simulink model "snap_sys_clk_feng"  (R2019a)
settings: Solver=VariableStepDiscrete  StartTime=0.0  StopTime=10.0  RelTol=1e-3
undefined symbols (not defined in the file): datetime, posixtime
libraries: xbsIndex_r4 x5252, casper_library_misc x69, xps_library x6, casper_library_delays x3
(part 1 of 45)
settings Model: Creator=jackh  LastModifiedBy=jackh
settings DataIOCC: ReturnWorkspaceOutputs=off
settings OptimizationCC: DefaultParameterBehavior=Inlined
settings DebuggingCC: ArithmeticOperatorsInVariantConditions=warning
settings SFSimCC: SimUseLocalCustomCode=off
settings RTWCC: RTWUseLocalCustomCode=off
settings CodeAppCC: StateflowObjectComments=on

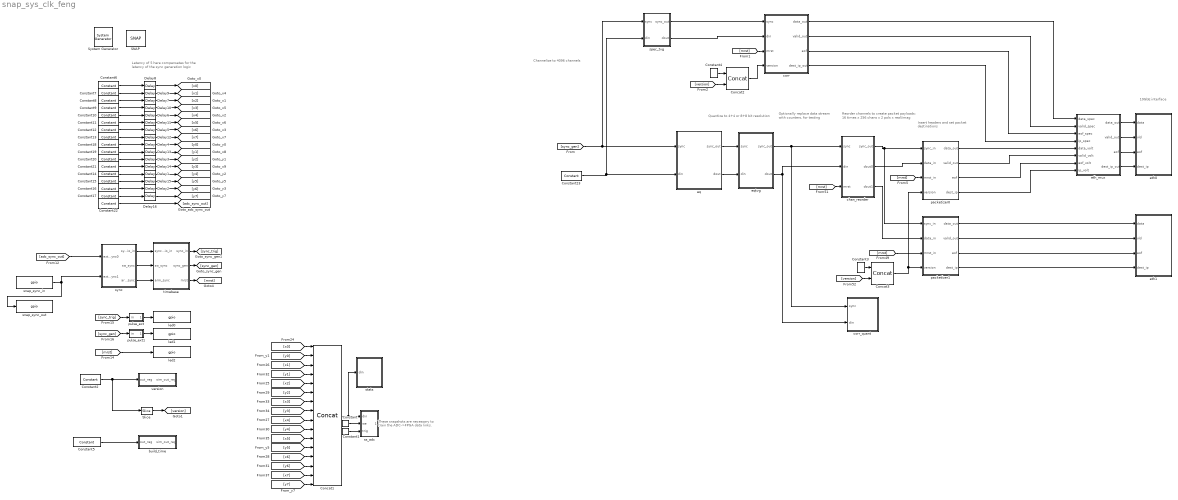
== system snap_sys_clk_feng ==
  note: 10GbE interface
  note: Insert headers and
      | set packet destinations
  note: Reorder channels to
      | create packet payloads:
      | 16 times x 256 chans x 2 pols x real/imag
  note: Optionally replace data
      | stream with counters, for testing
  note: Quantize to 4+4 or 8+8 bit resolution
  note: Channelize to 4096 channels
  note: These snapshots are necessary
      | to train the ADC->FPGA data links.
  note: Latency of 5 here compensates
      | for the latency of the sync generation logic
  " System Generator" : xbsIndex_r4/ System Generator  Tag=genX  xilinxfamily=kintex7  part=xc7k160t  speed=-2  package=ffg676  synthesis_tool=XST  clock_wrapper=Clock Enables  directory=/home/jackh/src/ata_snap/snap_sys_clk_feng/sysgen  proj_type=Vivado  Synth_file=Vivado Synthesis Defaults  Impl_file=Vivado Implementation Defaults  testbench=off  simulink_period=1  sysclk_period=10  dcm_input_clock_period=10  incr_netlist=off  trim_vbits=Everywhere in SubSystem  dbl_ovrd=According to Block Masks  core_generation=According to Block Masks  run_coregen=off  deprecated_control=off  eval_field=0  block_type=sysgen
  Concat1 : xbsIndex_r4/Concat  num_inputs=16  dbl_ovrd=off  block_type=concat
  Concat2 : xbsIndex_r4/Concat  num_inputs=2  dbl_ovrd=off  block_type=concat
  Concat3 : xbsIndex_r4/Concat  num_inputs=2  dbl_ovrd=off  block_type=concat
  Constant : xbsIndex_r4/Constant  const=0  gui_display_data_type=Boolean  arith_type=Boolean  n_bits=16  bin_pt=14  preci_type=Single  exp_width=8  frac_width=24  explicit_period=on  period=1  equ=P=C  opselect=C  inp2=PCIN>>17  opr=+  inp1=P  carry=CIN  dbl_ovrd=off  block_type=constant
  Constant1 : xbsIndex_r4/Constant  const=0  gui_display_data_type=Boolean  arith_type=Boolean  n_bits=16  bin_pt=14  preci_type=Single  exp_width=8  frac_width=24  explicit_period=on  period=1  equ=P=C  opselect=C  inp2=PCIN>>17  opr=+  inp1=P  carry=CIN  dbl_ovrd=off  block_type=constant
  Constant{6..21} (16 alike) : xbsIndex_r4/Constant  const=0  gui_display_data_type=Fixed-point  arith_type=Unsigned  n_bits=8  bin_pt=0  preci_type=Single  exp_width=8  frac_width=24  explicit_period=on  period=1  equ=P=C  opselect=C  inp2=PCIN>>17  opr=+  inp1=P  carry=CIN  dbl_ovrd=off  block_type=constant
  Constant2 : xbsIndex_r4/Constant  const=((2^6 + 2^5 + 0)*2^8) + 0  gui_display_data_type=Fixed-point  arith_type=Unsigned  n_bits=7+8  bin_pt=0  preci_type=Single  exp_width=8  frac_width=24  explicit_period=on  period=1  equ=P=C  opselect=C  inp2=PCIN>>17  opr=+  inp1=P  carry=CIN  dbl_ovrd=off  block_type=constant
  Constant22 : xbsIndex_r4/Constant  const=0  gui_display_data_type=Boolean  arith_type=Boolean  n_bits=8  bin_pt=7  preci_type=Single  exp_width=8  frac_width=24  explicit_period=on  period=1  equ=P=C  opselect=C  inp2=PCIN>>17  opr=+  inp1=P  carry=CIN  dbl_ovrd=off  block_type=constant
  Constant23 : xbsIndex_r4/Constant  const=0  gui_display_data_type=Fixed-point  arith_type=Unsigned  n_bits=400  bin_pt=0  preci_type=Single  exp_width=8  frac_width=24  explicit_period=on  period=1  equ=P=C  opselect=C  inp2=PCIN>>17  opr=+  inp1=P  carry=CIN  dbl_ovrd=off  block_type=constant
  Constant3 : xbsIndex_r4/Constant  const=1  gui_display_data_type=Fixed-point  arith_type=Unsigned  n_bits=1  bin_pt=0  preci_type=Single  exp_width=8  frac_width=24  explicit_period=on  period=1  equ=P=C  opselect=C  inp2=PCIN>>17  opr=+  inp1=P  carry=CIN  dbl_ovrd=off  block_type=constant
  Constant4 : xbsIndex_r4/Constant  const=0  gui_display_data_type=Fixed-point  arith_type=Unsigned  n_bits=1  bin_pt=0  preci_type=Single  exp_width=8  frac_width=24  explicit_period=on  period=1  equ=P=C  opselect=C  inp2=PCIN>>17  opr=+  inp1=P  carry=CIN  dbl_ovrd=off  block_type=constant
  Constant5 : xbsIndex_r4/Constant  const=int32(posixtime(datetime('now')))  gui_display_data_type=Fixed-point  arith_type=Unsigned  n_bits=32  bin_pt=0  preci_type=Single  exp_width=8  frac_width=24  explicit_period=on  period=1  equ=P=C  opselect=C  inp2=PCIN>>17  opr=+  inp1=P  carry=CIN  dbl_ovrd=off  block_type=constant
  Delay{1..16} (16 alike) : xbsIndex_r4/Delay  rst=off  infoeditControl=Selection of Reset will increase slice count due to use of real FFs and instead of SRLs  en=off  latency=5  reg_retiming=off  dbl_ovrd=off  block_type=delay
      settings: block_version=11.4
  SNAP : xps_library/Platforms/SNAP  Tag=xps:xsg  hw_sys=SNAP:xc7k160t  clk_src=sys_clk  clk_rate=100  use_microblaze=on  sample_period=1  synthesis_tool=XST
      settings: SourceProductName=CASPER XPS Blockset
  Slice : xbsIndex_r4/Slice  nbits=7  boolean_output=off  mode=Lower Bit Location + Width  bit1=0  base1=MSB of Input  bit0=8  base0=LSB of Input  dbl_ovrd=off  block_type=slice
  build_time : Subsystem  Tag=xps:sw_reg  AncestorBlock=xps_library/Memory/software_register  mask(swreg){io_dir=To Processor, io_delay=0, init_val=0, sample_period=1, names=reg, bitwidths=32, bin_pts=0, arith_types=0, sim_port=on, show_format=on}
      mask prompts: io_dir "I/O direction"; io_delay "I/O delay"; init_val "Initial Value"; sample_period "Sample period"; names "Bitfield names [msb...lsb]"; bitwidths "Bitfield widths"; bin_pts "Bitfield binary pts"; arith_types "Bitfield types, ufix=0, fix=1, bool=2"; sim_port "Provide sim input/output?"; show_format "Print format string?"
      mask help: A 32-bit software-accessible register. Can be divided into bitfields of varying widths and types using the fields in the block mask.
      mask init:
      | swreg_init(gcb)
      settings: AttributesFormatString=1output:uf32.0 = 32 bits
      mask TypeOptions io_dir: To Processor | From Processor
      mask Callback io_dir:
      | mask_enables = get_param(gcb, 'MaskEnables');
      | mask_names = get_param(gcb, 'MaskNames');
      | if strcmp(get_param(gcb, 'io_dir'), 'To Processor'),
      |     mask_enables{ismember(mask_names, 'sample_period')} = 'off';
      | else
      |     mask_enables{ismember(mask_names, 'sample_period')} = 'on';
      | end
      | set_param(gcb, 'MaskEnables', mask_enables);
      mask DialogControl ParameterTabVar0 Prompt: Setup
  chan_reorder : Subsystem
  corr : Subsystem  mask{n_chan_bits=12}
      mask prompts: n_chan_bits "Number of channels? (2^?)"
  corr_quant : Subsystem  mask{n_chan_bits=12}
      mask prompts: n_chan_bits "Number of channels? (2^?)"
  eq : Subsystem
  eqtvg : Subsystem
  eth0 : Subsystem
  eth1 : Subsystem
  eth_mux : Subsystem
  led0 : xps_library/IO/gpio  Tag=xps:gpio  io_group_params_forwarded=on  io_group=ROACH:led  io_group_real=led  io_group_custom=0  io_dir=out  arith_type=Boolean  bitwidth=1  bin_pt=0  bit_index=0  sample_period=1  use_single_ended=off  use_ddr=off  reg_iob=on  reg_clk_phase=0  termination=None
      settings: SourceProductName=CASPER XPS Blockset
  led1 : xps_library/IO/gpio  Tag=xps:gpio  io_group_params_forwarded=on  io_group=ROACH:led  io_group_real=led  io_group_custom=0  io_dir=out  arith_type=Boolean  bitwidth=1  bin_pt=0  bit_index=1  sample_period=1  use_single_ended=off  use_ddr=off  reg_iob=on  reg_clk_phase=0  termination=None
      settings: SourceProductName=CASPER XPS Blockset
  led2 : xps_library/IO/gpio  Tag=xps:gpio  io_group_params_forwarded=on  io_group=ROACH:led  io_group_real=led  io_group_custom=0  io_dir=out  arith_type=Boolean  bitwidth=1  bin_pt=0  bit_index=2  sample_period=1  use_single_ended=off  use_ddr=off  reg_iob=on  reg_clk_phase=0  termination=None
      settings: SourceProductName=CASPER XPS Blockset
  packetizer0 : Subsystem  mask{nchan_bits=12, npol_bits=4+1, nparallel_bits=3, step_bits=5, time_step_bits=4}
      mask prompts: nchan_bits "Number of channels (including unsent) (2^?)"; npol_bits "Number of pols (2^?)"; nparallel_bits "Parallel samples (2^?)"; step_bits "Step granularity (2^?)"; time_step_bits "Time Steps per cycle (2^?)"
  packetizer1 : Subsystem  mask{nchan_bits=12, npol_bits=4+1, nparallel_bits=3, step_bits=5, time_step_bits=4}
      mask prompts: nchan_bits "Number of channels (including unsent) (2^?)"; npol_bits "Number of pols (2^?)"; nparallel_bits "Parallel samples (2^?)"; step_bits "Step granularity (2^?)"; time_step_bits "Time Steps per cycle (2^?)"
  pulse_ext : Subsystem  AncestorBlock=casper_library_misc/pulse_ext  mask(pulse_ext){pulse_len=2^25}
      mask prompts: pulse_len "Length of Pulse"
      mask help:
      | Extends a boolean signal to be high for the specified number of clocks after
      | the last high input.
      mask init:
      | bits = ceil(log2(pulse_len+1));
      mask Help: eval('xlWeb(''http://casper.berkeley.edu/wiki/Pulse_ext'')')
  pulse_ext1 : Subsystem  AncestorBlock=casper_library_misc/pulse_ext  mask(pulse_ext){pulse_len=2^25}
      mask prompts: pulse_len "Length of Pulse"
      mask help:
      | Extends a boolean signal to be high for the specified number of clocks after
      | the last high input.
      mask init:
      | bits = ceil(log2(pulse_len+1));
      mask Help: eval('xlWeb(''http://casper.berkeley.edu/wiki/Pulse_ext'')')
  snap_sync_in : xps_library/IO/gpio  Tag=xps:gpio  io_group_params_forwarded=on  io_group=ROACH:led  io_group_real=sync_in  io_group_custom=0  io_dir=in  arith_type=Boolean  bitwidth=1  bin_pt=0  bit_index=0  sample_period=1  use_single_ended=off  use_ddr=off  reg_iob=on  reg_clk_phase=0  termination=None
      settings: SourceProductName=CASPER XPS Blockset
  snap_sync_out : xps_library/IO/gpio  Tag=xps:gpio  io_group_params_forwarded=on  io_group=ROACH:led  io_group_real=sync_out  io_group_custom=0  io_dir=out  arith_type=Boolean  bitwidth=1  bin_pt=0  bit_index=0  sample_period=1  use_single_ended=on  use_ddr=off  reg_iob=on  reg_clk_phase=0  termination=None
      settings: SourceProductName=CASPER XPS Blockset
  spec_tvg : Subsystem
  ss_adc : Subsystem  Tag=casper:snapshot  AncestorBlock=casper_library_scopes/snapshot  mask(snapshot){storage=bram, dram_dimm=1, dram_clock=200, nsamples=9, data_width=128, offset=off, circap=off, value=off, ext_arm=off, ext_circ=off, provide_outputs=on, use_dsp48=off}
      mask prompts: storage "Storage medium"; dram_dimm "DRAM dimm"; dram_clock "DRAM clock rate"; nsamples "Number of Samples (2^?)"; data_width "Data width"; offset "Start delay support"; circap "Circular capture support"; value "Extra value capture support"; ext_arm "External arm support"; ext_circ "External circular capture support"; provide_outputs "Provide outputs"; use_dsp48 "Use DSP48s to implement counters"
      mask help:
      | Standard snap block, but with the following optional extras;
      |  1) Optionally delay the fabric trigger by a user-specified number of valids.
      |  2) Capture continuously after a trigger until a stop pulse is received. Data is captured into BRAM continuously, with old data being overwritten until a stop command is received. Then stop capturing when memory is filled. This enables you to get some data before and some data after the stop pulse. Use the 'tr_en_cnt' register to determine where you are in your vector. 'Addr' register's MSb now indicates 'busy capturing'.
      |  3) Optionally capture a value on an input port to a register at the same time as the first data sample.
      |  4) Implement counters using DSP48Es to save resources.
      mask init:
      | snapshot_init(gcb, ...
      |     'storage', storage, ...
      |     'dram_dimm', dram_dimm, ...
      |     'dram_clock', dram_clock, ...
      |     'nsamples', nsamples, ...
      |     'data_width', data_width, ...
      |     'offset', offset, ...
      |     'circap', circap, ...
      |     'value', value, ...
      |     'ext_arm', ext_arm, ...
      |     'ext_circ', ext_circ, ...
      |     'provide_outputs', 'off', ...
      |     'use_dsp48', use_dsp48);
      settings: AttributesFormatString=|
      | 128 wide, 512 deep
      | debugID: 6419356
      mask TypeOptions storage: bram | dram
      mask Callback storage: snapshot_callback();
      mask TypeOptions dram_dimm: 1 | 2 | 3 | 4
      mask TypeOptions dram_clock: 200 | 250 | 266 | 300 | 333
      mask TypeOptions data_width: 8 | 16 | 32 | 64 | 128
  stats : Subsystem
  sync : Subsystem
  timebase : Subsystem
  version : Subsystem  Tag=xps:sw_reg  AncestorBlock=xps_library/Memory/software_register  mask(swreg){io_dir=To Processor, io_delay=0, init_val=0, sample_period=1, names=reg, bitwidths=7+8, bin_pts=0, arith_types=0, sim_port=on, show_format=on}
      mask prompts: io_dir "I/O direction"; io_delay "I/O delay"; init_val "Initial Value"; sample_period "Sample period"; names "Bitfield names [msb...lsb]"; bitwidths "Bitfield widths"; bin_pts "Bitfield binary pts"; arith_types "Bitfield types, ufix=0, fix=1, bool=2"; sim_port "Provide sim input/output?"; show_format "Print format string?"
      mask help: A 32-bit software-accessible register. Can be divided into bitfields of varying widths and types using the fields in the block mask.
      mask init:
      | swreg_init(gcb)
      settings: AttributesFormatString=1output:uf15.0 = 15 bits
      mask TypeOptions io_dir: To Processor | From Processor
      mask Callback io_dir:
      | mask_enables = get_param(gcb, 'MaskEnables');
      | mask_names = get_param(gcb, 'MaskNames');
      | if strcmp(get_param(gcb, 'io_dir'), 'To Processor'),
      |     mask_enables{ismember(mask_names, 'sample_period')} = 'off';
      | else
      |     mask_enables{ismember(mask_names, 'sample_period')} = 'on';
      | end
      | set_param(gcb, 'MaskEnables', mask_enables);
      mask DialogControl ParameterTabVar0 Prompt: Setup
  wires:
  sync/1(sync_gpio_in) -> timebase/1(sync_gpio_in)
  sync/2(sw_sync) -> timebase/2(sw_sync)
  sync/3(arm_sync) -> timebase/3(arm_sync)
  timebase/2(sync_gen) -> [sync_gen]
  timebase/1(sync_in) -> [sync_trig]
  timebase/3(mrst) -> [mrst]
  [adc_sync_out] -> sync/1(ext_sync0)
  [mrst] -> led2/1
  pulse_ext/1(out) -> led0/1
  pulse_ext1/1(out) -> led1/1
  [sync_trig] -> pulse_ext/1(in)
  [sync_gen] -> pulse_ext1/1(in)
  Delay2/1 -> [y6]
  Delay1/1 -> [y4]
  Delay3/1 -> [y2]
  Delay4/1 -> [y0]
  Delay5/1 -> [x6]
  Delay6/1 -> [x4]
  Delay7/1 -> [x2]
  Delay8/1 -> [x0]
  Concat1/1 -> stats/1(din), ss_adc/1(din)
  Constant/1 -> ss_adc/2(we)
  Constant1/1 -> ss_adc/3(trig)
  Delay9/1 -> [x1]
  Delay10/1 -> [x3]
  Delay11/1 -> [x5]
  Delay12/1 -> [x7]
  Delay13/1 -> [y1]
  Delay14/1 -> [y3]
  Delay15/1 -> [y5]
  Delay16/1 -> [y7]
  [x0] -> Concat1/1
  [y0] -> Concat1/2
  [x2] -> Concat1/5
  [y2] -> Concat1/6
  [x4] -> Concat1/9
  [y4] -> Concat1/10
  [x6] -> Concat1/13
  [x1] -> Concat1/3
  [y1] -> Concat1/4
  [x3] -> Concat1/7
  [y3] -> Concat1/8
  [x5] -> Concat1/11
  [y5] -> Concat1/12
  [y6] -> Concat1/14
  [x7] -> Concat1/15
  [y7] -> Concat1/16
  Constant23/1 -> spec_tvg/2(din), eq/2(din)
  [sync_gen] -> spec_tvg/1(sync), eq/1(sync)
  eq/1(sync_out) -> eqtvg/1(sync)
  eq/2(dout) -> eqtvg/2(din)
  eqtvg/1(sync_out) -> chan_reorder/1(sync), corr_quant/1(sync)
  eqtvg/2(dout) -> chan_reorder/2(din), corr_quant/2(din)
  chan_reorder/1(sync_out) -> packetizer1/1(sync_in), packetizer0/1(sync_in)
  chan_reorder/2(dout0) -> packetizer0/2(data_in)
  [mrst] -> corr/3(mrst)
  corr/1(data_out) -> eth_mux/1(data_spec)
  corr/2(valid_out) -> eth_mux/2(valid_spec)
  corr/3(eof) -> eth_mux/3(eof_spec)
  corr/4(dest_ip_out) -> eth_mux/4(ip_spec)
  eth_mux/1(data_out) -> eth0/1(data)
  eth_mux/2(valid_out) -> eth0/2(vld)
  eth_mux/3(eof) -> eth0/3(eof)
  eth_mux/4(dest_ip_out) -> eth0/4(dest_ip)
  Constant2/1 -> version/1(out_reg), Slice/1
  Slice/1 -> [version]
  Constant4/1 -> Concat2/1
  [version] -> Concat2/2
  Concat2/1 -> corr/4(version)
  spec_tvg/1(sync_out) -> corr/1(sync)
  spec_tvg/2(dout) -> corr/2(din)
  Constant6/1 -> Delay8/1
  Constant7/1 -> Delay9/1
  Constant8/1 -> Delay7/1
  Constant9/1 -> Delay10/1
  Constant10/1 -> Delay6/1
  Constant11/1 -> Delay11/1
  Constant12/1 -> Delay5/1
  Constant13/1 -> Delay12/1
  Constant18/1 -> Delay4/1
  Constant19/1 -> Delay13/1
  Constant20/1 -> Delay3/1
  Constant21/1 -> Delay14/1
  Constant14/1 -> Delay1/1
  Constant15/1 -> Delay15/1
  Constant16/1 -> Delay2/1
  Constant17/1 -> Delay16/1
  Constant22/1 -> [adc_sync_out]
  snap_sync_in/1 -> snap_sync_out/1, sync/2(ext_sync1)
  Constant5/1 -> build_time/1(out_reg)
  [mrst] -> chan_reorder/3(mrst)
  packetizer0/1(data_out) -> eth_mux/5(data_volt)
  packetizer0/2(valid_out) -> eth_mux/6(valid_volt)
  packetizer0/3(eof) -> eth_mux/7(eof_volt)
  packetizer0/4(dest_ip) -> eth_mux/8(ip_volt)
  [mrst] -> packetizer0/3(mrst_in)
  Concat3/1 -> packetizer1/4(version), packetizer0/4(version)
  packetizer1/1(data_out) -> eth1/1(data)
  packetizer1/2(valid_out) -> eth1/2(vld)
  packetizer1/3(eof) -> eth1/3(eof)
  packetizer1/4(dest_ip) -> eth1/4(dest_ip)
  [mrst] -> packetizer1/3(mrst_in)
  chan_reorder/3(dout1) -> packetizer1/2(data_in)
  Constant3/1 -> Concat3/1
  [version] -> Concat3/2

== system snap_sys_clk_feng/build_time ==
  out_reg : Inport
  assert_reg : xbsIndex_r4/Assert  assert_type=on  type_source=Explicitly  gui_display_data_type=Fixed-point  arith_type=Unsigned  n_bits=32  bin_pt=0  preci_type=Single  exp_width=8  frac_width=24  assert_rate=off  rate_source=Explicitly  period=1  output_port=on  block_type=assert
  cast_gw : xbsIndex_r4/Convert  gui_display_data_type=Fixed-point  arith_type=Unsigned  n_bits=32  bin_pt=0  float_type=Single  exp_bits=8  fraction_bits=24  quantization=Truncate  overflow=Wrap  en=off  latency=1  pipeline=off  dbl_ovrd=off  block_type=convert
  io_delay : xbsIndex_r4/Delay  rst=off  infoeditControl=Selection of Reset will increase slice count due to use of real FFs and instead of SRLs  en=off  latency=0  reg_retiming=on  dbl_ovrd=off  block_type=delay
  reint1 : xbsIndex_r4/Reinterpret  force_arith_type=on  arith_type=Unsigned  force_bin_pt=on  bin_pt=0  block_type=reinterpret
  sim_out : Terminator
  sim_out_reg_gw : xbsIndex_r4/Gateway Out  inherit_from_input=off  hdl_port=off  rows=1  columns=1  UseAsDAC=off  DACChannel='1'  interface=None  automatic_assignment=on  address_offset=hex2dec('00')  intf_name=''  intf_description=''  timing_constraint=None  locs_specified=off  LOCs={}  io_standard={}  block_type=gatewayout
  sim_out_reg_sim_delay : xbsIndex_r4/Delay  rst=off  infoeditControl=Selection of Reset will increase slice count due to use of real FFs and instead of SRLs  en=off  latency=1  reg_retiming=on  dbl_ovrd=off  block_type=delay
  snap_sys_clk_feng_build_time_user_data_in : xbsIndex_r4/Gateway Out  inherit_from_input=off  hdl_port=on  rows=1  columns=1  UseAsDAC=off  DACChannel='1'  interface=None  automatic_assignment=on  address_offset=hex2dec('00')  intf_name=''  intf_description=''  timing_constraint=None  locs_specified=off  LOCs={}  io_standard={}  block_type=gatewayout
  sim_out_reg : Outport
  wires:
  sim_out_reg_sim_delay/1 -> sim_out_reg_gw/1
  sim_out_reg_gw/1 -> sim_out_reg/1
  io_delay/1 -> cast_gw/1
  cast_gw/1 -> snap_sys_clk_feng_build_time_user_data_in/1
  snap_sys_clk_feng_build_time_user_data_in/1 -> sim_out/1
  out_reg/1 -> sim_out_reg_sim_delay/1, assert_reg/1
  assert_reg/1 -> reint1/1
  reint1/1 -> io_delay/1

== system snap_sys_clk_feng/chan_reorder ==
  note: in 4-bit mode -- slice the bits we care about
      | and send them to both packetizers.
      |
      | in 8 bit mode, split frequencies
  note: Only allow one sync after MRST.
      | This is because we don't know the appropriate
      | reorder orders for non-double-buffered runtime-configuratble
      | reorders
  note: input: 16 times x 1024 chans x 4 chans(parallel) x 2 pols
      |
      | output:
      | 1024 chans x 16 times x 4 chans (parallel) x 2 pols
      |
      | OR
      |
      | Nc x 16 times x 1024/Nc chans x 4 chans (parallel) x 2 pols
  note: reorder serial channels
      | so channels which we don't care about
      | can be placed in convenient
      | place to facilitate inter-packet gaps
  note: Reorder each parallel 64 bits to combine polarizations:
      |
      | order is now:
      |
      | serial_chans (1024) x parallel_chans (4) x pols (2)
  note: Use this programmable
      | map to mess with the channel
      | ordering.
      |
      | This lets us interleave channels we want to send, with channels
      | we don't care about, allowing the data rate to be kept below 10Gb/s
      |
      | Input is 4 channels x 2 pols in parallel.
      | Over 1024 clocks we get a full spectrum for these inputs.
  note: output:
      | 4096 chans x 4 times x 4 time (parallel) x 2 pols
  sync : Inport
  din : Inport  Port=2
  mrst : Inport  Port=3
  Constant4 : xbsIndex_r4/Constant  const=1.0  gui_display_data_type=Boolean  arith_type=Boolean  n_bits=16  bin_pt=14  preci_type=Single  exp_width=8  frac_width=24  explicit_period=on  period=1  equ=P=C  opselect=C  inp2=PCIN>>17  opr=+  inp1=P  carry=CIN  dbl_ovrd=off  block_type=constant
  Delay : xbsIndex_r4/Delay  rst=off  infoeditControl=Selection of Reset will increase slice count due to use of real FFs and instead of SRLs  en=off  latency=1  reg_retiming=off  dbl_ovrd=off  block_type=delay
  Delay1 : xbsIndex_r4/Delay  rst=off  infoeditControl=Selection of Reset will increase slice count due to use of real FFs and instead of SRLs  en=off  latency=1  reg_retiming=off  dbl_ovrd=off  block_type=delay
  Delay2 : xbsIndex_r4/Delay  rst=off  infoeditControl=Selection of Reset will increase slice count due to use of real FFs and instead of SRLs  en=off  latency=1  reg_retiming=off  dbl_ovrd=off  block_type=delay
  Inverter : xbsIndex_r4/Inverter  en=off  latency=0  dbl_ovrd=off  block_type=inv
  Logical : xbsIndex_r4/Logical  logical_function=AND  inputs=2  en=off  latency=0  precision=Full  arith_type=Unsigned  n_bits=16  bin_pt=0  align_bp=on  dbl_ovrd=off  block_type=logical
  Mux2 : xbsIndex_r4/Mux  inputs=2  en=off  latency=1  precision=Full  arith_type=Unsigned  n_bits=16  bin_pt=14  quantization=Truncate  overflow=Wrap  dbl_ovrd=off  block_type=mux
  Mux3 : xbsIndex_r4/Mux  inputs=2  en=off  latency=1  precision=Full  arith_type=Unsigned  n_bits=16  bin_pt=14  quantization=Truncate  overflow=Wrap  dbl_ovrd=off  block_type=mux
  Mux5 : xbsIndex_r4/Mux  inputs=2  en=off  latency=1  precision=Full  arith_type=Unsigned  n_bits=16  bin_pt=14  quantization=Truncate  overflow=Wrap  dbl_ovrd=off  block_type=mux
  Register : xbsIndex_r4/Register  init=0  rst=on  en=on  dbl_ovrd=off  block_type=register
  demux : Subsystem
  gpu_weird_order : Subsystem  Tag=xps:sw_reg  AncestorBlock=xps_library/Memory/software_register  mask(swreg){io_dir=From Processor, io_delay=0, init_val=0, sample_period=1, names=reg, bitwidths=1, bin_pts=0, arith_types=0, sim_port=on, show_format=on}
      mask prompts: io_dir "I/O direction"; io_delay "I/O delay"; init_val "Initial Value"; sample_period "Sample period"; names "Bitfield names [msb...lsb]"; bitwidths "Bitfield widths"; bin_pts "Bitfield binary pts"; arith_types "Bitfield types, ufix=0, fix=1, bool=2"; sim_port "Provide sim input/output?"; show_format "Print format string?"
      mask help: A 32-bit software-accessible register. Can be divided into bitfields of varying widths and types using the fields in the block mask.
      mask init:
      | swreg_init(gcb)
      settings: AttributesFormatString=1input:uf1.0 = 1 bits
      mask TypeOptions io_dir: To Processor | From Processor
      mask Callback io_dir:
      | mask_enables = get_param(gcb, 'MaskEnables');
      | mask_names = get_param(gcb, 'MaskNames');
      | if strcmp(get_param(gcb, 'io_dir'), 'To Processor'),
      |     mask_enables{ismember(mask_names, 'sample_period')} = 'off';
      | else
      |     mask_enables{ismember(mask_names, 'sample_period')} = 'on';
      | end
      | set_param(gcb, 'MaskEnables', mask_enables);
      mask DialogControl ParameterTabVar0 Prompt: Setup
  parallel_reorder1 : Subsystem
  reorder3 : Subsystem  AncestorBlock=casper_library_reorder/reorder  mask(reorder){map=reshape(permute(reshape([0:1024*16 - 1], 1024, 16), [2,1]), 1024*16, 1), n_bits=2*4*16, n_inputs=1, bram_latency=2, map_latency=2, fanout_latency=2, double_buffer=0, bram_map=on, software_controlled=off}
      mask prompts: map "Output Order:"; n_bits "Data width in"; n_inputs "Number of inputs"; bram_latency "BRAM Latency"; map_latency "Map Latency"; fanout_latency "Fanout latency"; double_buffer "Double Buffer"; bram_map "Use BlockRAM for Map"; software_controlled "Use runtime software control"
      mask init:
      | reorder_init(gcb, ...
      |     'map', map, ...
      |     'n_bits', n_bits, ...
      |     'n_inputs', n_inputs, ...
      |     'bram_latency', bram_latency, ...
      |     'map_latency', map_latency, ...
      |     'fanout_latency', fanout_latency, ...
      |     'double_buffer', double_buffer, ...
      |     'bram_map', bram_map, ...
      |     'software_controlled', software_controlled);
      settings: AttributesFormatString=order=7
      mask Help: eval('xlWeb(''http://casper.berkeley.edu/wiki/Reorder'')')
  skip_c_t_transpose : Subsystem  Tag=xps:sw_reg  AncestorBlock=xps_library/Memory/software_register  mask(swreg){io_dir=From Processor, io_delay=0, init_val=0, sample_period=1, names=reg, bitwidths=1, bin_pts=0, arith_types=0, sim_port=on, show_format=on}
      mask prompts: io_dir "I/O direction"; io_delay "I/O delay"; init_val "Initial Value"; sample_period "Sample period"; names "Bitfield names [msb...lsb]"; bitwidths "Bitfield widths"; bin_pts "Bitfield binary pts"; arith_types "Bitfield types, ufix=0, fix=1, bool=2"; sim_port "Provide sim input/output?"; show_format "Print format string?"
      mask help: A 32-bit software-accessible register. Can be divided into bitfields of varying widths and types using the fields in the block mask.
      mask init:
      | swreg_init(gcb)
      settings: AttributesFormatString=1input:uf1.0 = 1 bits
      mask TypeOptions io_dir: To Processor | From Processor
      mask Callback io_dir:
      | mask_enables = get_param(gcb, 'MaskEnables');
      | mask_names = get_param(gcb, 'MaskNames');
      | if strcmp(get_param(gcb, 'io_dir'), 'To Processor'),
      |     mask_enables{ismember(mask_names, 'sample_period')} = 'off';
      | else
      |     mask_enables{ismember(mask_names, 'sample_period')} = 'on';
      | end
      | set_param(gcb, 'MaskEnables', mask_enables);
      mask DialogControl ParameterTabVar0 Prompt: Setup
  slice_duplicate : Subsystem
  transpose_t_c : Subsystem
  use_8bit : Subsystem  Tag=xps:sw_reg  AncestorBlock=xps_library/Memory/software_register  mask(swreg){io_dir=From Processor, io_delay=0, init_val=0, sample_period=1, names=reg, bitwidths=1, bin_pts=0, arith_types=0, sim_port=on, show_format=on}
      mask prompts: io_dir "I/O direction"; io_delay "I/O delay"; init_val "Initial Value"; sample_period "Sample period"; names "Bitfield names [msb...lsb]"; bitwidths "Bitfield widths"; bin_pts "Bitfield binary pts"; arith_types "Bitfield types, ufix=0, fix=1, bool=2"; sim_port "Provide sim input/output?"; show_format "Print format string?"
      mask help: A 32-bit software-accessible register. Can be divided into bitfields of varying widths and types using the fields in the block mask.
      mask init:
      | swreg_init(gcb)
      settings: AttributesFormatString=1input:uf1.0 = 1 bits
      mask TypeOptions io_dir: To Processor | From Processor
      mask Callback io_dir:
      | mask_enables = get_param(gcb, 'MaskEnables');
      | mask_names = get_param(gcb, 'MaskNames');
      | if strcmp(get_param(gcb, 'io_dir'), 'To Processor'),
      |     mask_enables{ismember(mask_names, 'sample_period')} = 'off';
      | else
      |     mask_enables{ismember(mask_names, 'sample_period')} = 'on';
      | end
      | set_param(gcb, 'MaskEnables', mask_enables);
      mask DialogControl ParameterTabVar0 Prompt: Setup
  sync_out : Outport
  dout0 : Outport  Port=2
  dout1 : Outport  Port=3
  wires:
  din/1 -> parallel_reorder1/1(din)
  sync/1 -> Logical/2, Register/1, Register/3
  Logical/1 -> reorder3/1(sync)
  Constant4/1 -> reorder3/2(en)
  parallel_reorder1/1(dout) -> reorder3/3(din0)
  Mux2/1 -> dout0/1
  mrst/1 -> Register/2
  Register/1 -> Inverter/1
  Inverter/1 -> Logical/1
  Mux3/1 -> dout1/1
  use_8bit/1(in_reg) -> Delay2/1, Delay1/1, Delay/1
  Mux5/1 -> sync_out/1
  reorder3/1(sync_out) -> transpose_t_c/1(sync)
  reorder3/3(dout0) -> transpose_t_c/2(din)
  transpose_t_c/1(sync_out) -> slice_duplicate/1(sync), demux/1(sync)
  transpose_t_c/2(dout) -> demux/2(din), slice_duplicate/2(din)
  slice_duplicate/1(sync_out) -> [sync_4bit]
  slice_duplicate/2(dout0) -> [d0_4bit]
  slice_duplicate/3(dout1) -> [d1_4bit]
  demux/1(sync_out) -> [sync_8bit]
  demux/2(dout0) -> [d0_8bit]
  demux/3(dout1) -> [d1_8bit]
  [sync_4bit] -> Mux5/2
  [sync_8bit] -> Mux5/3
  [d1_4bit] -> Mux3/2
  [d1_8bit] -> Mux3/3
  [d0_4bit] -> Mux2/2
  [d0_8bit] -> Mux2/3
  Delay/1 -> Mux3/1
  Delay1/1 -> Mux2/1
  Delay2/1 -> Mux5/1
  skip_c_t_transpose/1(in_reg) -> transpose_t_c/3(bypass)
  gpu_weird_order/1(in_reg) -> slice_duplicate/3(gpu_order)

== system snap_sys_clk_feng/corr ==
  sync : Inport
  din : Inport  Port=2
  mrst : Inport  Port=3
  version : Inport  Port=4
  bus_expand : Subsystem  AncestorBlock=casper_library_flow_control/bus_expand  mask(bus_expand){mode=divisions of equal size, outputNum=2, outputWidth=25*2*4, outputBinaryPt=0, outputArithmeticType=0, show_format=off, outputToWorkspace=off, variablePrefix=out, outputToModelAsWell=on}
      mask prompts: outputNum "Number of outputs:"; outputWidth "Output width:"; outputBinaryPt "Output binary point position:"; outputArithmeticType "Output arithmetic type (ufix=0, fix=1, bool=2):"; show_format "Print format string?"; outputToWorkspace "Output to workspace?"; variablePrefix "Variable name prefix:"; outputToModelAsWell "Output to model as well?"
      mask help:
      | Expands a 'bus' made using a bus_create or Xilinx
      | concat block.
      | The input will be divided into the specified number
      | of outputs with the specified arithmetic types.
      | Divisions are made from most significant bit.
      mask init:
      | bus_expand_init(gcb,...
      |     'mode', mode, ...
      |     'outputNum', outputNum, ...
      |     'outputWidth', outputWidth, ...
      |     'outputBinaryPt', outputBinaryPt, ...
      |     'outputArithmeticType', outputArithmeticType, ...
      |     'show_format', show_format, ...
      |     'outputToWorkspace', outputToWorkspace, ...
      |     'variablePrefix', variablePrefix, ...
      |     'outputToModelAsWell', outputToModelAsWell);
      settings: AttributesFormatString=2 outputs
      mask TypeOptions mode: divisions of equal size | divisions of arbitrary size
      mask Callback mode: bus_expand_callback();
      mask Callback outputWidth: bus_expand_callback();
      mask Callback outputToWorkspace: bus_expand_callback();
  bus_expand1 : Subsystem  AncestorBlock=casper_library_flow_control/bus_expand  mask(bus_expand){mode=divisions of equal size, outputNum=4, outputWidth=25*2, outputBinaryPt=0, outputArithmeticType=1, show_format=off, outputToWorkspace=off, variablePrefix=out, outputToModelAsWell=on}
      mask prompts: outputNum "Number of outputs:"; outputWidth "Output width:"; outputBinaryPt "Output binary point position:"; outputArithmeticType "Output arithmetic type (ufix=0, fix=1, bool=2):"; show_format "Print format string?"; outputToWorkspace "Output to workspace?"; variablePrefix "Variable name prefix:"; outputToModelAsWell "Output to model as well?"
      mask help:
      | Expands a 'bus' made using a bus_create or Xilinx
      | concat block.
      | The input will be divided into the specified number
      | of outputs with the specified arithmetic types.
      | Divisions are made from most significant bit.
      mask init: same as snap_sys_clk_feng/corr/bus_expand
      settings: AttributesFormatString=4 outputs
      mask TypeOptions mode: divisions of equal size | divisions of arbitrary size
      mask Callback mode: bus_expand_callback();
      mask Callback outputWidth: bus_expand_callback();
      mask Callback outputToWorkspace: bus_expand_callback();
  bus_expand2 : Subsystem  AncestorBlock=casper_library_flow_control/bus_expand  mask(bus_expand){mode=divisions of equal size, outputNum=4, outputWidth=25*2, outputBinaryPt=0, outputArithmeticType=1, show_format=off, outputToWorkspace=off, variablePrefix=out, outputToModelAsWell=on}
      mask prompts: outputNum "Number of outputs:"; outputWidth "Output width:"; outputBinaryPt "Output binary point position:"; outputArithmeticType "Output arithmetic type (ufix=0, fix=1, bool=2):"; show_format "Print format string?"; outputToWorkspace "Output to workspace?"; variablePrefix "Variable name prefix:"; outputToModelAsWell "Output to model as well?"
      mask help:
      | Expands a 'bus' made using a bus_create or Xilinx
      | concat block.
      | The input will be divided into the specified number
      | of outputs with the specified arithmetic types.
      | Divisions are made from most significant bit.
      mask init: same as snap_sys_clk_feng/corr/bus_expand
      settings: AttributesFormatString=4 outputs
      mask TypeOptions mode: divisions of equal size | divisions of arbitrary size
      mask Callback mode: bus_expand_callback();
      mask Callback outputWidth: bus_expand_callback();
      mask Callback outputToWorkspace: bus_expand_callback();
  bus_expand3 : Subsystem  AncestorBlock=casper_library_flow_control/bus_expand  mask(bus_expand){mode=divisions of equal size, outputNum=4, outputWidth=25*2, outputBinaryPt=0, outputArithmeticType=1, show_format=off, outputToWorkspace=off, variablePrefix=out, outputToModelAsWell=on}
      mask prompts: outputNum "Number of outputs:"; outputWidth "Output width:"; outputBinaryPt "Output binary point position:"; outputArithmeticType "Output arithmetic type (ufix=0, fix=1, bool=2):"; show_format "Print format string?"; outputToWorkspace "Output to workspace?"; variablePrefix "Variable name prefix:"; outputToModelAsWell "Output to model as well?"
      mask help:
      | Expands a 'bus' made using a bus_create or Xilinx
      | concat block.
      | The input will be divided into the specified number
      | of outputs with the specified arithmetic types.
      | Divisions are made from most significant bit.
      mask init: same as snap_sys_clk_feng/corr/bus_expand
      settings: AttributesFormatString=4 outputs
      mask TypeOptions mode: divisions of equal size | divisions of arbitrary size
      mask Callback mode: bus_expand_callback();
      mask Callback outputWidth: bus_expand_callback();
      mask Callback outputToWorkspace: bus_expand_callback();
  bus_expand4 : Subsystem  AncestorBlock=casper_library_flow_control/bus_expand  mask(bus_expand){mode=divisions of equal size, outputNum=4, outputWidth=25*2, outputBinaryPt=0, outputArithmeticType=1, show_format=off, outputToWorkspace=off, variablePrefix=out, outputToModelAsWell=on}
      mask prompts: outputNum "Number of outputs:"; outputWidth "Output width:"; outputBinaryPt "Output binary point position:"; outputArithmeticType "Output arithmetic type (ufix=0, fix=1, bool=2):"; show_format "Print format string?"; outputToWorkspace "Output to workspace?"; variablePrefix "Variable name prefix:"; outputToModelAsWell "Output to model as well?"
      mask help:
      | Expands a 'bus' made using a bus_create or Xilinx
      | concat block.
      | The input will be divided into the specified number
      | of outputs with the specified arithmetic types.
      | Divisions are made from most significant bit.
      mask init: same as snap_sys_clk_feng/corr/bus_expand
      settings: AttributesFormatString=4 outputs
      mask TypeOptions mode: divisions of equal size | divisions of arbitrary size
      mask Callback mode: bus_expand_callback();
      mask Callback outputWidth: bus_expand_callback();
      mask Callback outputToWorkspace: bus_expand_callback();
  crosspower_vacc : Subsystem  mask{bw=25, nchan=2^n_chan_bits, vacc_bw=64, vacc_bp=48}
      mask prompts: bw "Bitwidth in"; nchan "Number of channels"; vacc_bw "Vector accumulator output bitwidth"; vacc_bp "Vector accumulator output binary point"
  dest_ip : Subsystem  Tag=xps:sw_reg  AncestorBlock=xps_library/Memory/software_register  mask(swreg){io_dir=From Processor, io_delay=0, init_val=0, sample_period=1, names=reg, bitwidths=32, bin_pts=0, arith_types=0, sim_port=on, show_format=on}
      mask prompts: io_dir "I/O direction"; io_delay "I/O delay"; init_val "Initial Value"; sample_period "Sample period"; names "Bitfield names [msb...lsb]"; bitwidths "Bitfield widths"; bin_pts "Bitfield binary pts"; arith_types "Bitfield types, ufix=0, fix=1, bool=2"; sim_port "Provide sim input/output?"; show_format "Print format string?"
      mask help: A 32-bit software-accessible register. Can be divided into bitfields of varying widths and types using the fields in the block mask.
      mask init:
      | swreg_init(gcb)
      settings: AttributesFormatString=1input:uf32.0 = 32 bits
      mask TypeOptions io_dir: To Processor | From Processor
      mask Callback io_dir:
      | mask_enables = get_param(gcb, 'MaskEnables');
      | mask_names = get_param(gcb, 'MaskNames');
      | if strcmp(get_param(gcb, 'io_dir'), 'To Processor'),
      |     mask_enables{ismember(mask_names, 'sample_period')} = 'off';
      | else
      |     mask_enables{ismember(mask_names, 'sample_period')} = 'on';
      | end
      | set_param(gcb, 'MaskEnables', mask_enables);
      mask DialogControl ParameterTabVar0 Prompt: Setup
  feng_id : Subsystem  Tag=xps:sw_reg  AncestorBlock=xps_library/Memory/software_register  mask(swreg){io_dir=From Processor, io_delay=0, init_val=0, sample_period=1, names=reg, bitwidths=8, bin_pts=0, arith_types=0, sim_port=on, show_format=on}
      mask prompts: io_dir "I/O direction"; io_delay "I/O delay"; init_val "Initial Value"; sample_period "Sample period"; names "Bitfield names [msb...lsb]"; bitwidths "Bitfield widths"; bin_pts "Bitfield binary pts"; arith_types "Bitfield types, ufix=0, fix=1, bool=2"; sim_port "Provide sim input/output?"; show_format "Print format string?"
      mask help: A 32-bit software-accessible register. Can be divided into bitfields of varying widths and types using the fields in the block mask.
      mask init:
      | swreg_init(gcb)
      settings: AttributesFormatString=1input:uf8.0 = 8 bits
      mask TypeOptions io_dir: To Processor | From Processor
      mask Callback io_dir:
      | mask_enables = get_param(gcb, 'MaskEnables');
      | mask_names = get_param(gcb, 'MaskNames');
      | if strcmp(get_param(gcb, 'io_dir'), 'To Processor'),
      |     mask_enables{ismember(mask_names, 'sample_period')} = 'off';
      | else
      |     mask_enables{ismember(mask_names, 'sample_period')} = 'on';
      | end
      | set_param(gcb, 'MaskEnables', mask_enables);
      mask DialogControl ParameterTabVar0 Prompt: Setup
  power_vacc0 : Subsystem  mask{bw=25, nchan=2^n_chan_bits, vacc_bw=64, vacc_bp=48}
      mask prompts: bw "Bitwidth in"; nchan "Number of channels"; vacc_bw "Vector accumulator output bitwidth"; vacc_bp "Vector accumulator output binary point"
  power_vacc1 : Subsystem  mask{bw=25, nchan=2^n_chan_bits, vacc_bw=64, vacc_bp=48}
      mask prompts: bw "Bitwidth in"; nchan "Number of channels"; vacc_bw "Vector accumulator output bitwidth"; vacc_bp "Vector accumulator output binary point"
  vacc_output : Subsystem
  vacc_ss : Subsystem  mask{n_chan_bits=n_chan_bits}
      mask prompts: n_chan_bits "Number of channels (2^?)"
      mask init:
      | ss0 = [gcb '/ss0']
      | ss1 = [gcb '/ss1']
      | 
      | nsamples = num2str(n_chan_bits - 2);
      | 
      | set_param(ss0, 'nsamples', nsamples);
      | set_param(ss1, 'nsamples', nsamples);
  data_out : Outport
  valid_out : Outport  Port=2
  eof : Outport  Port=3
  dest_ip_out : Outport  Port=4
  wires:
  [sync_in] -> power_vacc0/1(new_acc)
  power_vacc0/1(vld) -> [vacc_vld]
  din/1 -> bus_expand/1(bus_in)
  bus_expand/1(msb_out2) -> [x]
  bus_expand/2(lsb_out1) -> [y]
  [x] -> bus_expand1/1(bus_in)
  [sync_in] -> power_vacc1/1(new_acc)
  sync/1 -> [sync_in]
  [y] -> bus_expand2/1(bus_in)
  [mrst_in] -> vacc_output/1(rst)
  [xx_0] -> vacc_ss/2(xx0)
  [vacc_vld] -> vacc_ss/1(vld)
  [xx_1] -> vacc_ss/3(xx1)
  [vacc_vld] -> vacc_output/14(vld)
  mrst/1 -> [mrst_in]
  power_vacc0/2(out0) -> [xx_0]
  power_vacc0/3(out1) -> [xx_1]
  power_vacc0/4(out2) -> [xx_2]
  power_vacc0/5(out3) -> [xx_3]
  power_vacc1/2(out0) -> [yy_0]
  power_vacc1/3(out1) -> [yy_1]
  power_vacc1/4(out2) -> [yy_2]
  power_vacc1/5(out3) -> [yy_3]
  [x] -> bus_expand3/1(bus_in)
  [sync_in] -> crosspower_vacc/1(new_acc)
  [y] -> bus_expand4/1(bus_in)
  crosspower_vacc/2(xy0) -> [xy_0]
  crosspower_vacc/5(xy3) -> [xy_3]
  crosspower_vacc/4(xy2) -> [xy_2]
  crosspower_vacc/3(xy1) -> [xy_1]
  [xx_2] -> vacc_ss/4(xx2)
  [xx_3] -> vacc_ss/5(xx3)
  [yy_0] -> vacc_ss/6(yy0)
  [yy_1] -> vacc_ss/7(yy1)
  [yy_2] -> vacc_ss/8(yy2)
  [yy_3] -> vacc_ss/9(yy3)
  [xy_0] -> vacc_ss/10(xy0)
  [xy_1] -> vacc_ss/11(xy1)
  [xy_2] -> vacc_ss/12(xy2)
  [xy_3] -> vacc_ss/13(xy3)
  [xx_0] -> vacc_output/2(xx0)
  [xx_1] -> vacc_output/3(xx1)
  [xx_2] -> vacc_output/4(xx2)
  [xx_3] -> vacc_output/5(xx3)
  [yy_0] -> vacc_output/6(yy0)
  [yy_1] -> vacc_output/7(yy1)
  [yy_2] -> vacc_output/8(yy2)
  [yy_3] -> vacc_output/9(yy3)
  [xy_0] -> vacc_output/10(xy0)
  [xy_1] -> vacc_output/11(xy1)
  [xy_2] -> vacc_output/12(xy2)
  [xy_3] -> vacc_output/13(xy3)
  vacc_output/3(eof) -> eof/1
  dest_ip/1(in_reg) -> dest_ip_out/1
  vacc_output/1(dout) -> data_out/1
  vacc_output/2(vld_out) -> valid_out/1
  version/1 -> vacc_output/15(version)
  feng_id/1(in_reg) -> vacc_output/16(ant_id)
  bus_expand1/1(msb_out4) -> power_vacc0/2(in0)
  bus_expand1/2(out3) -> power_vacc0/3(in1)
  bus_expand1/3(out2) -> power_vacc0/4(in2)
  bus_expand1/4(lsb_out1) -> power_vacc0/5(in3)
  bus_expand2/1(msb_out4) -> power_vacc1/2(in0)
  bus_expand2/2(out3) -> power_vacc1/3(in1)
  bus_expand2/3(out2) -> power_vacc1/4(in2)
  bus_expand2/4(lsb_out1) -> power_vacc1/5(in3)
  bus_expand3/1(msb_out4) -> crosspower_vacc/2(x0)
  bus_expand3/2(out3) -> crosspower_vacc/3(x1)
  bus_expand3/3(out2) -> crosspower_vacc/4(x2)
  bus_expand3/4(lsb_out1) -> crosspower_vacc/5(x3)
  bus_expand4/1(msb_out4) -> crosspower_vacc/6(y0)
  bus_expand4/2(out3) -> crosspower_vacc/7(y1)
  bus_expand4/3(out2) -> crosspower_vacc/8(y2)
  bus_expand4/4(lsb_out1) -> crosspower_vacc/9(y3)

== system snap_sys_clk_feng/corr_quant ==
  sync : Inport
  din : Inport  Port=2
  bus_expand : Subsystem  AncestorBlock=casper_library_flow_control/bus_expand  mask(bus_expand){mode=divisions of equal size, outputNum=2, outputWidth=4*2*8, outputBinaryPt=0, outputArithmeticType=0, show_format=off, outputToWorkspace=off, variablePrefix=out, outputToModelAsWell=on}
      mask prompts: outputNum "Number of outputs:"; outputWidth "Output width:"; outputBinaryPt "Output binary point position:"; outputArithmeticType "Output arithmetic type (ufix=0, fix=1, bool=2):"; show_format "Print format string?"; outputToWorkspace "Output to workspace?"; variablePrefix "Variable name prefix:"; outputToModelAsWell "Output to model as well?"
      mask help:
      | Expands a 'bus' made using a bus_create or Xilinx
      | concat block.
      | The input will be divided into the specified number
      | of outputs with the specified arithmetic types.
      | Divisions are made from most significant bit.
      mask init: same as snap_sys_clk_feng/corr/bus_expand
      settings: AttributesFormatString=2 outputs
      mask TypeOptions mode: divisions of equal size | divisions of arbitrary size
      mask Callback mode: bus_expand_callback();
      mask Callback outputWidth: bus_expand_callback();
      mask Callback outputToWorkspace: bus_expand_callback();
  bus_expand1 : Subsystem  AncestorBlock=casper_library_flow_control/bus_expand  mask(bus_expand){mode=divisions of equal size, outputNum=4, outputWidth=8*2, outputBinaryPt=0, outputArithmeticType=1, show_format=off, outputToWorkspace=off, variablePrefix=out, outputToModelAsWell=on}
      mask prompts: outputNum "Number of outputs:"; outputWidth "Output width:"; outputBinaryPt "Output binary point position:"; outputArithmeticType "Output arithmetic type (ufix=0, fix=1, bool=2):"; show_format "Print format string?"; outputToWorkspace "Output to workspace?"; variablePrefix "Variable name prefix:"; outputToModelAsWell "Output to model as well?"
      mask help:
      | Expands a 'bus' made using a bus_create or Xilinx
      | concat block.
      | The input will be divided into the specified number
      | of outputs with the specified arithmetic types.
      | Divisions are made from most significant bit.
      mask init: same as snap_sys_clk_feng/corr/bus_expand
      settings: AttributesFormatString=4 outputs
      mask TypeOptions mode: divisions of equal size | divisions of arbitrary size
      mask Callback mode: bus_expand_callback();
      mask Callback outputWidth: bus_expand_callback();
      mask Callback outputToWorkspace: bus_expand_callback();
  bus_expand2 : Subsystem  AncestorBlock=casper_library_flow_control/bus_expand  mask(bus_expand){mode=divisions of equal size, outputNum=4, outputWidth=8*2, outputBinaryPt=0, outputArithmeticType=1, show_format=off, outputToWorkspace=off, variablePrefix=out, outputToModelAsWell=on}
      mask prompts: outputNum "Number of outputs:"; outputWidth "Output width:"; outputBinaryPt "Output binary point position:"; outputArithmeticType "Output arithmetic type (ufix=0, fix=1, bool=2):"; show_format "Print format string?"; outputToWorkspace "Output to workspace?"; variablePrefix "Variable name prefix:"; outputToModelAsWell "Output to model as well?"
      mask help:
      | Expands a 'bus' made using a bus_create or Xilinx
      | concat block.
      | The input will be divided into the specified number
      | of outputs with the specified arithmetic types.
      | Divisions are made from most significant bit.
      mask init: same as snap_sys_clk_feng/corr/bus_expand
      settings: AttributesFormatString=4 outputs
      mask TypeOptions mode: divisions of equal size | divisions of arbitrary size
      mask Callback mode: bus_expand_callback();
      mask Callback outputWidth: bus_expand_callback();
      mask Callback outputToWorkspace: bus_expand_callback();
  power_vacc0 : Subsystem  mask{bw=8, nchan=2^n_chan_bits, vacc_bw=32, vacc_bp=14}
      mask prompts: bw "Bitwidth in"; nchan "Number of channels"; vacc_bw "Vector accumulator output bitwidth"; vacc_bp "Vector accumulator output binary point"
  power_vacc1 : Subsystem  mask{bw=8, nchan=2^n_chan_bits, vacc_bw=32, vacc_bp=14}
      mask prompts: bw "Bitwidth in"; nchan "Number of channels"; vacc_bw "Vector accumulator output bitwidth"; vacc_bp "Vector accumulator output binary point"
  vacc_ss : Subsystem  mask{n_chan_bits=n_chan_bits}
      mask prompts: n_chan_bits "Number of channels (2^?)"
      mask init:
      | ss0 = [gcb '/ss0']
      | %ss1 = [gcb '/ss1']
      | 
      | nsamples = num2str(n_chan_bits - 2);
      | 
      | set_param(ss0, 'nsamples', nsamples);
      | %set_param(ss1, 'nsamples', nsamples);
  wires:
  bus_expand2/4(lsb_out1) -> power_vacc1/5(in3)
  bus_expand2/3(out2) -> power_vacc1/4(in2)
  bus_expand2/2(out3) -> power_vacc1/3(in1)
  bus_expand2/1(msb_out4) -> power_vacc1/2(in0)
  bus_expand1/4(lsb_out1) -> power_vacc0/5(in3)
  bus_expand1/3(out2) -> power_vacc0/4(in2)
  bus_expand1/2(out3) -> power_vacc0/3(in1)
  bus_expand1/1(msb_out4) -> power_vacc0/2(in0)
  [yy_3] -> vacc_ss/9(yy3)
  [yy_2] -> vacc_ss/8(yy2)
  [yy_1] -> vacc_ss/7(yy1)
  [yy_0] -> vacc_ss/6(yy0)
  [xx_3] -> vacc_ss/5(xx3)
  [xx_2] -> vacc_ss/4(xx2)
  power_vacc1/5(out3) -> [yy_3]
  power_vacc1/4(out2) -> [yy_2]
  power_vacc1/3(out1) -> [yy_1]
  power_vacc1/2(out0) -> [yy_0]
  power_vacc0/5(out3) -> [xx_3]
  power_vacc0/4(out2) -> [xx_2]
  power_vacc0/3(out1) -> [xx_1]
  power_vacc0/2(out0) -> [xx_0]
  [xx_1] -> vacc_ss/3(xx1)
  [vacc_vld] -> vacc_ss/1(vld)
  [xx_0] -> vacc_ss/2(xx0)
  [y] -> bus_expand2/1(bus_in)
  sync/1 -> [sync_in]
  [sync_in] -> power_vacc1/1(new_acc)
  [x] -> bus_expand1/1(bus_in)
  bus_expand/2(lsb_out1) -> [y]
  bus_expand/1(msb_out2) -> [x]
  din/1 -> bus_expand/1(bus_in)
  power_vacc0/1(vld) -> [vacc_vld]
  [sync_in] -> power_vacc0/1(new_acc)
